simulink model "TSetup2023a"  (R2023a)
settings: Solver=ode4  StartTime=0.0  StopTime=inf  FixedStep=0.01  RelTol=1e-3
libraries: AFCToolbox x3
settings Model: Creator=zqinghua  LastModifiedBy=zqhkd
settings OptimizationCC: DefaultParameterBehavior=Inlined  EnhancedBackFolding=on  PassReuseOutputArgsAs=Individual arguments  ZeroExternalMemoryAtStartup=off  ZeroInternalMemoryAtStartup=off  OptimizeBlockOrder=speed  DifferentSizesBufferReuse=on  OptimizationCustomize=off  EfficientTunableParamExpr=on
settings DebuggingCC: ParameterTunabilityLossMsg=error
settings HardwareCC: ProdBitPerInt=16  ProdBitPerPointer=16  ProdBitPerSizeT=16  ProdBitPerPtrDiffT=16  ProdLargestAtomicFloat=None  ProdWordSize=16  ProdHWDeviceType=STMicroelectronics->ST10/Super10
settings SFSimCC: MATLABDynamicMemAlloc=off
settings RTWCC: Description=Embedded Coder  SystemTargetFile=AFCHawk.tlc  GenCodeOnly=on  TemplateMakefile=ert_default_tmf
settings CodeAppCC: ForceParamTrailComments=on  IgnoreCustomStorageClasses=off  OperatorAnnotations=on  SimulinkDataObjDesc=on  SFDataObjDesc=on  InsertBlockDesc=on
settings STFCustomTargetCC: MultiwordLength=256  ModelReferenceCompliant=off  ConcurrentExecutionCompliant=off  CombineOutputUpdateFcns=on  ERTCustomFileBanners=on  SupportContinuousTime=off  SupportNonInlinedSFcns=off  RemoveResetFunc=on  MATLABClassNameForMDSCustomization=Simulink.SoftwareTarget.ERTCustomization  GRTInterface=off  UseToolchainInfoCompliant=off  SystemTargetFile=AFCHawk.tlc
settings ERTTargetCC: TargetLangStandard=C99 (ISO)  ModelReferenceCompliant=off  ParMdlRefBuildCompliant=off  CompOptLevelCompliant=off  ConcurrentExecutionCompliant=off  ModelStepFunctionPrototypeControlCompliant=off  CPPClassGenCompliant=off  UseToolchainInfoCompliant=off  InlinedParameterPlacement=NonHierarchical  ERTCustomFileTemplate=example_file_process.tlc
settings ConfigComp: CovBoundaryAbsTol=1.0e-5

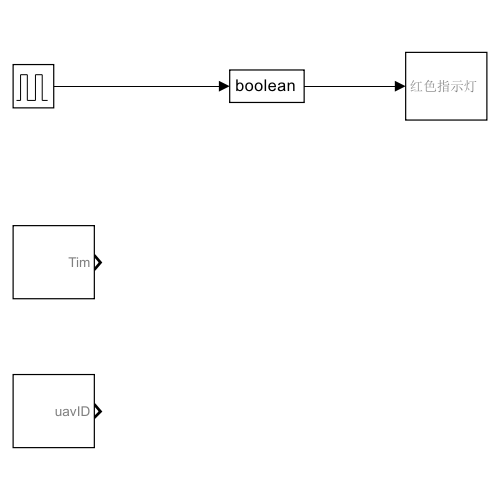
[thumbnail: Simulink's stored preview of the top-level diagram]
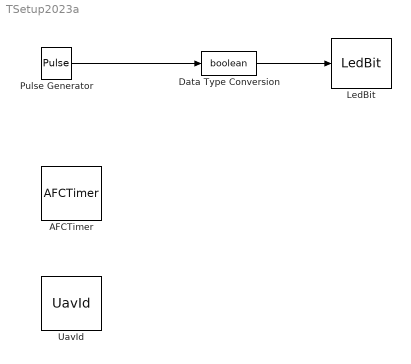
== system TSetup2023a ==
  AFCTimer : AFCToolbox/DeviceModule/AFCTimer  Priority=0  g_sampleTime=0.01  g_comPort=6  g_instName=0  g_id=0
      settings: SourceProductName=AFCToolbox
  Data Type Conversion : DataTypeConversion  OutDataTypeStr=boolean  SaturateOnIntegerOverflow=off  RndMeth=Floor
  LedBit : AFCToolbox/DeviceModule/LedBit  Priority=6  g_chanelNo=红色指示灯  g_comPort=0  g_instName=0  g_id=0
      settings: SourceProductName=AFCToolbox
  Pulse Generator : DiscretePulseGenerator  PulseType=Time based  Period=1  PulseWidth=30
  UavId : AFCToolbox/DeviceModule/UavId  Priority=0  g_sampleTime=0.01  g_comPort=6  g_instName=0  g_id=0
      settings: SourceProductName=AFCToolbox
  wires:
  Pulse Generator/1 -> Data Type Conversion/1
  Data Type Conversion/1 -> LedBit/1
